simulink model "FlightGearInterface_Example"  (R2018b)
settings: Solver=FixedStepAuto  StartTime=0.0  StopTime=inf  FixedStep=0.030  RelTol=1e-3
libraries: flightgear_visualization_lib x1
settings Model: EnablePacing=on  Creator=fabian  LastModifiedBy=yannic

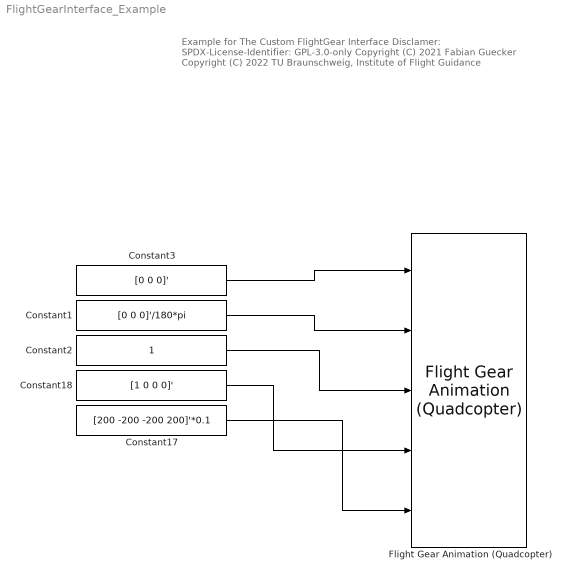
== system FlightGearInterface_Example ==
  note: Example for The Custom FlightGear Interface
      |
      | Disclamer:
      | SPDX-License-Identifier: GPL-3.0-only
      |
      | Copyright (C) 2021 Fabian Guecker
      | Copyright (C) 2022 TU Braunschweig, Institute of Flight Guidance
  Constant1 : Constant  Value=[0 0 0]'/180*pi  VectorParams1D=off
  Constant17 : Constant  Value=[200 -200 -200 200]'*0.1  VectorParams1D=off
  Constant18 : Constant  Value=[1 0 0 0]'  VectorParams1D=off
  Constant2 : Constant
  Constant3 : Constant  Value=[0 0 0]'  VectorParams1D=off
  Flight Gear Animation (Quadcopter) : flightgear_visualization_lib/Flight Gear Animation (Quadcopter)  inital_lat=37.616540510056176  inital_long=-122.36460730785899  inital_height=20  remoteURL='127.0.0.1'  remotePort=5502
      settings: SourceProductName=LADAC
  wires:
  Constant3/1 -> Flight Gear Animation (Quadcopter)/1
  Constant1/1 -> Flight Gear Animation (Quadcopter)/2
  Constant2/1 -> Flight Gear Animation (Quadcopter)/3
  Constant18/1 -> Flight Gear Animation (Quadcopter)/4
  Constant17/1 -> Flight Gear Animation (Quadcopter)/5
